simulink model "ControladorMathworksPX4"  (R2026a)
settings: Solver=FixedStepDiscrete  StopTime=1
PreLoadFcn:
  | InitVars;
values from neighbouring files (symbols this model uses):
  ArmConstants = struct('l1_dim', l1_dim,                        'l2_dim', l2_dim,                        'Hexa_to_joint_L', L,                        'Mass1', ml1,                        'Mass2', ml2,                        'Inertia1', Hl1,                        'Inertia2', Hl2,                        'MC1', c1,                        'MC2', c2,                        'Servos', Servos)    [init_model.m]    (also in init_var.m)
libraries: px4uORBlib x4, px4Peripheralslib x1, sharedutil x1, sharedtransform x1
settings Model: ExtModeTrigDuration=10  Creator=The MathWorks, Inc.  LastModifiedBy=Carlos Fabian
settings SolverCC: PositivePriorityOrder=on
settings OptimizationCC: UseDivisionForNetSlopeComputation=on  GainParamInheritBuiltInType=on  UseFloatMulNetSlope=on  InlineInvariantSignals=on  NoFixptDivByZeroProtection=on  EfficientFloat2IntCast=on  LifeSpan=1
settings HardwareCC: ProdLargestAtomicInteger=Long  ProdLargestAtomicFloat=Double  ProdHWDeviceType=ARM Compatible->ARM Cortex
settings SFSimCC: SimTargetLang=C++
settings RTWCC: SystemTargetFile=ert.tlc  HardwareBoard=PX4 Host Target  TLCOptions="-aInlineSetEventsForThisBaseRateFcn=TLC_FALSE -aSuppressMultiTaskScheduler=TLC_FALSE  -aRateBasedStepFcn=0"  GenCodeOnly=on  Toolchain=GNU Tools for PX4 Autopilots  PortableWordSizes=on  TargetLang=C++  Description=Embedded Coder
settings ERTTargetCC: ExtModeTransport=2.0  RootIOFormat=Structure reference  ERTFilePackagingFormat=CompactWithDataFile  DynamicArrayContainerType=coder::array  IncludeMdlTerminateFcn=off  CombineSignalStateStructs=on  CodeInterfacePackaging=Reusable function  SupportComplex=off

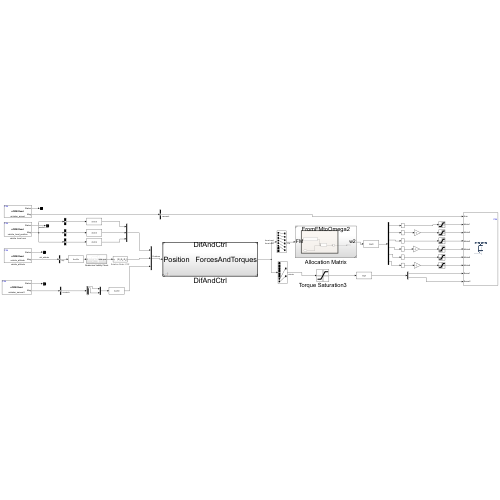
[thumbnail: Simulink's stored preview of the top-level diagram]
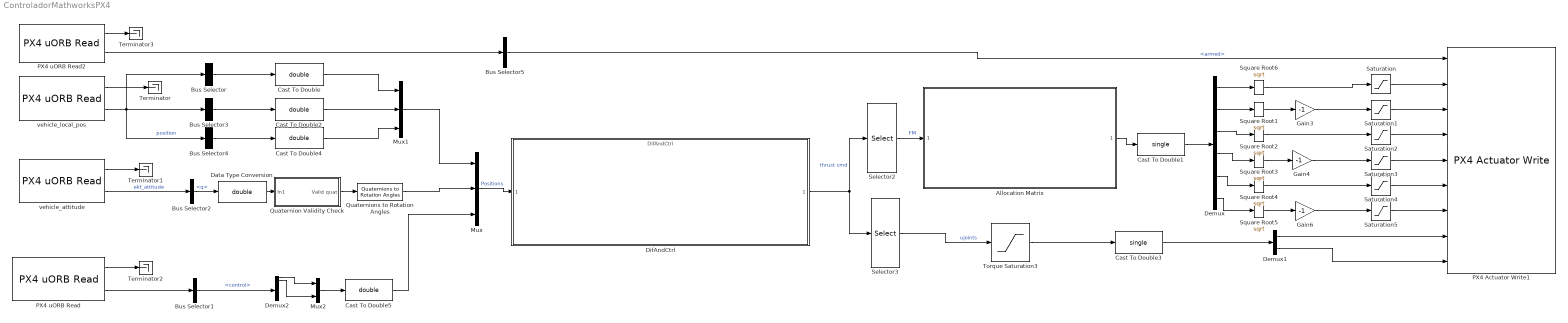
== system ControladorMathworksPX4 ==
  Allocation Matrix : Subsystem  ReferencedSubsystem=FromFMtoOmega2
  Bus Selector : BusSelector  OutputSignals=x  OutputAsBus=on
  Bus Selector1 : BusSelector  OutputSignals=control
  Bus Selector2 : BusSelector  OutputSignals=q
  Bus Selector3 : BusSelector  OutputSignals=y  OutputAsBus=on
  Bus Selector4 : BusSelector  OutputSignals=z  OutputAsBus=on
  Bus Selector5 : BusSelector  OutputSignals=armed
  Cast To Double{,2,4..5} (4 alike) : DataTypeConversion  OutDataTypeStr=double  SaturateOnIntegerOverflow=off  RndMeth=Floor
  Cast To Double1 : DataTypeConversion  OutDataTypeStr=single  SaturateOnIntegerOverflow=off  RndMeth=Floor
  Cast To Double3 : DataTypeConversion  OutDataTypeStr=single  SaturateOnIntegerOverflow=off  RndMeth=Floor
  Data Type Conversion : DataTypeConversion  OutDataTypeStr=double  SaturateOnIntegerOverflow=off  RndMeth=Floor
  Demux : Demux  Outputs=6
  Demux1 : Demux  Outputs=2
  Demux2 : Demux  Outputs=8
  DifAndCtrl : ModelReference  ModelNameDialog=DifAndCtrl  SimulationMode=Normal  ModelReferenceVersion=1.86
  Gain3 : Gain  Gain=-1
  Gain4 : Gain  Gain=-1
  Gain6 : Gain  Gain=-1
  Mux : Mux  Inputs=3
  Mux1 : Mux  Inputs=3
  Mux2 : Mux  Inputs=2
  PX4 Actuator Write1 : px4Peripheralslib/PX4 Actuator Write  Motor1Enable=on  Motor2Enable=on  Motor3Enable=on  Motor4Enable=on  Motor5Enable=on  Motor6Enable=on  Motor7Enable=off  Motor8Enable=off  Motor9Enable=off  Motor10Enable=off  Motor11Enable=off  Motor12Enable=off  IsMotorArray=off  Servo1Enable=on  Servo2Enable=on  Servo3Enable=off  Servo4Enable=off  Servo5Enable=off  Servo6Enable=off  Servo7Enable=off  Servo8Enable=off  IsServoArray=off
  PX4 uORB Read : px4uORBlib/PX4 uORB Read  uORBMsg=ActuatorServos  uORBTopicName=actuator_servos  SubscribeNonZeroInstance=on  selectInstanceNum=2  SampleTime=0.01  isSingleTopicMsg=on  BlockingMode=off  BlockTimeout=1e-3
  PX4 uORB Read2 : px4uORBlib/PX4 uORB Read  uORBMsg=ActuatorArmed  uORBTopicName=actuator_armed  SubscribeNonZeroInstance=off  selectInstanceNum=1  SampleTime=-1  isSingleTopicMsg=on  BlockingMode=off  BlockTimeout=1e-3
  Quaternion Validity Check : Subsystem
  Quaternions to Rotation Angles : sharedtransform/Quaternions to Rotation Angles  rotationOrder=XYZ  aMode=aMode
  Saturation{,1..5} (6 alike) : Saturate  UpperLimit=1  LowerLimit=-1
  Selector2 : Selector  InputPortWidth=8  IndexOptions=Index vector (dialog)  Indices=1:6  OutputSizes=1
  Selector3 : Selector  InputPortWidth=8  IndexOptions=Index vector (dialog)  Indices=7:8  OutputSizes=1
  Square Root{1..6} (6 alike) : Sqrt
  Terminator{,1..3} (4 alike) : Terminator
  Torque Saturation3 : Saturate  UpperLimit=ArmConstants.Servos.T1max  LowerLimit=-ArmConstants.Servos.T1max
  vehicle_attitude : px4uORBlib/PX4 uORB Read  uORBMsg=VehicleAttitude  uORBTopicName=vehicle_attitude  SubscribeNonZeroInstance=off  selectInstanceNum=1  SampleTime=0.01  isSingleTopicMsg=off  BlockingMode=off  BlockTimeout=1e-3
  vehicle_local_pos : px4uORBlib/PX4 uORB Read  uORBMsg=VehicleLocalPosition  uORBTopicName=vehicle_local_position  SubscribeNonZeroInstance=off  selectInstanceNum=1  SampleTime=0.01  isSingleTopicMsg=off  BlockingMode=off  BlockTimeout=1e-3
  wires:
  Mux/1 -> DifAndCtrl/1  "Positions"
  Torque Saturation3/1 -> Cast To Double3/1
  Square Root2/1 -> Saturation2/1
  Cast To Double3/1 -> Demux1/1
  Demux1/1 -> PX4 Actuator Write1/8
  Selector2/1 -> Allocation Matrix/1  "FM"
  Saturation1/1 -> PX4 Actuator Write1/3
  Demux/3 -> Square Root2/1
  Selector3/1 -> Torque Saturation3/1  "ujoints"
  Saturation3/1 -> PX4 Actuator Write1/5
  Gain3/1 -> Saturation1/1
  Allocation Matrix/1 -> Cast To Double1/1
  Demux1/2 -> PX4 Actuator Write1/9
  Square Root3/1 -> Gain4/1
  Demux/2 -> Square Root1/1
  Square Root4/1 -> Saturation4/1
  Demux/4 -> Square Root3/1
  Demux/1 -> Square Root6/1
  Gain4/1 -> Saturation3/1
  Demux/6 -> Square Root5/1
  Gain6/1 -> Saturation5/1
  Square Root1/1 -> Gain3/1
  Cast To Double1/1 -> Demux/1
  Square Root5/1 -> Gain6/1
  DifAndCtrl/1 -> Selector2/1, Selector3/1  "thrust cmd"
  Saturation4/1 -> PX4 Actuator Write1/6
  Saturation5/1 -> PX4 Actuator Write1/7
  Saturation2/1 -> PX4 Actuator Write1/4
  Demux/5 -> Square Root4/1
  Square Root6/1 -> Saturation/1
  Saturation/1 -> PX4 Actuator Write1/2
  Cast To Double/1 -> Mux1/1
  Data Type Conversion/1 -> Quaternion Validity Check/1(In1)
  vehicle_attitude/1 -> Terminator1/1
  Cast To Double4/1 -> Mux1/3
  Bus Selector3/1 -> Cast To Double2/1
  vehicle_local_pos/2 -> Bus Selector/1, Bus Selector4/1, Bus Selector3/1  "position"
  vehicle_attitude/2 -> Bus Selector2/1  "ekf_attitude"
  Quaternion Validity Check/1(Valid quat) -> Quaternions to Rotation Angles/1
  PX4 uORB Read2/1 -> Terminator3/1
  PX4 uORB Read/2 -> Bus Selector1/1
  Bus Selector5/1 -> PX4 Actuator Write1/1  "<armed>"
  Demux2/1 -> Mux2/1
  vehicle_local_pos/1 -> Terminator/1
  PX4 uORB Read/1 -> Terminator2/1
  PX4 uORB Read2/2 -> Bus Selector5/1
  Bus Selector1/1 -> Demux2/1  "<control>"
  Bus Selector2/1 -> Data Type Conversion/1  "<q>"
  Cast To Double5/1 -> Mux/3
  Demux2/2 -> Mux2/2
  Bus Selector/1 -> Cast To Double/1
  Mux1/1 -> Mux/1
  Mux2/1 -> Cast To Double5/1
  Cast To Double2/1 -> Mux1/2
  Bus Selector4/1 -> Cast To Double4/1
  Quaternions to Rotation Angles/1 -> Mux/2

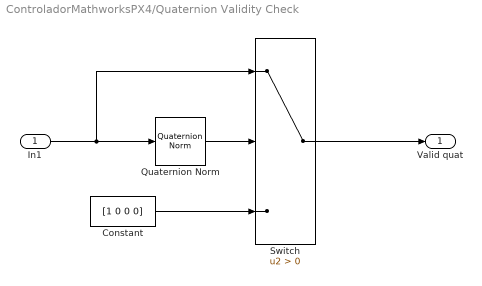
== system ControladorMathworksPX4/Quaternion Validity Check ==
  In1 : Inport
  Constant : Constant  Value=[1 0 0 0]  SampleTime=-1
  Quaternion Norm : sharedutil/Quaternion Norm  aMode=aMode
  Switch : Switch  Criteria=u2 > Threshold  SaturateOnIntegerOverflow=off  InputSameDT=off
  Valid quat : Outport
  wires:
  In1/1 -> Quaternion Norm/1, Switch/1
  Quaternion Norm/1 -> Switch/2
  Switch/1 -> Valid quat/1
  Constant/1 -> Switch/3
